simulink model "sim_tanque"  (R2025b)
settings: Solver=VariableStepAuto  StartTime=0.0  StopTime=10.0  RelTol=1e-3
values from neighbouring files (symbols this model uses):
  A = 0.5    [Aula08_lab.m]    (also in Lab10.m; Lab5_6.m; lab3.m; lab4.m)
  g = 9.8    [Aula08_lab.m]    (also in Lab10.m; Lab5_6.m; lab3.m; lab4.m)
  H0 = ((ke*ae0)/(ks*as0*sqrt(2*g)))^2    [Aula08_lab.m]    (also in Lab10.m; Lab5_6.m; lab3.m = H_eq; lab4.m = ((Ke .* ae0) ./ (Ks .* as0 .* sqrt(2*g))).^2)
  Ke = 0.05    [lab3.m]    (also in lab4.m; lab4_bonitinho.m)
  Ks = 0.015    [lab3.m]    (also in lab4.m; lab4_bonitinho.m)
undefined symbols (not defined in the file or in its folder): Ae, As

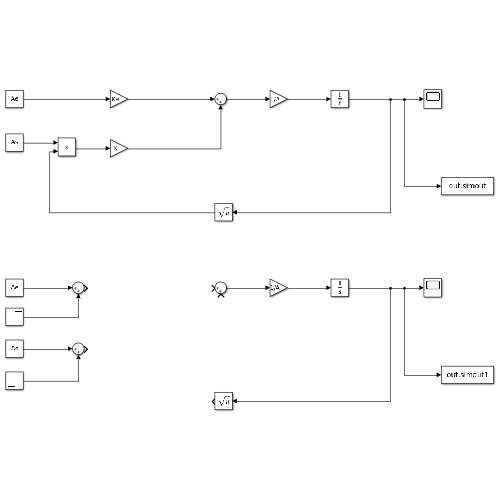
[thumbnail: Simulink's stored preview of the top-level diagram]
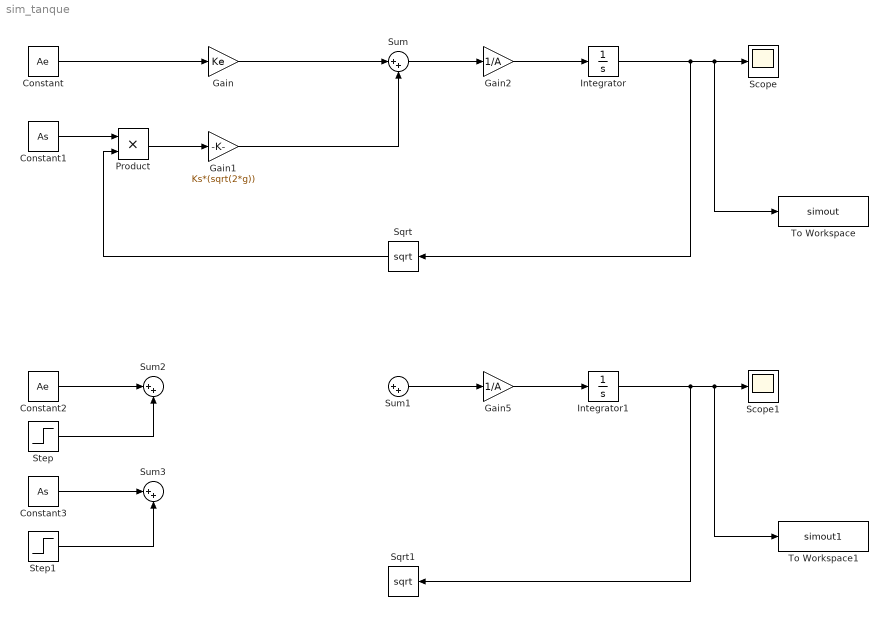
== system sim_tanque ==
  Constant : Constant  Value=Ae
  Constant1 : Constant  Value=As
  Constant2 : Constant  Value=Ae
  Constant3 : Constant  Value=As
  Gain : Gain  Gain=Ke
  Gain1 : Gain  Gain=Ks*(sqrt(2*g))
  Gain2 : Gain  Gain=1/A
  Gain5 : Gain  Gain=1/A
  Integrator : Integrator  InitialCondition=H0
  Integrator1 : Integrator
  Product : Product
  Scope : Scope
  Scope1 : Scope
  Sqrt : Sqrt
  Sqrt1 : Sqrt
  Step : Step  SampleTime=0
  Step1 : Step  SampleTime=0
  Sum{,1..3} (4 alike) : Sum  Inputs=|++
  To Workspace : ToWorkspace  VariableName=simout  SaveFormat=Timeseries  SampleTime=-1
  To Workspace1 : ToWorkspace  VariableName=simout1  SaveFormat=Timeseries  SampleTime=-1
  wires:
  Constant/1 -> Gain/1
  Gain/1 -> Sum/1
  Sum/1 -> Gain2/1
  Gain2/1 -> Integrator/1
  Integrator/1 -> Sqrt/1, To Workspace/1, Scope/1
  Constant1/1 -> Product/1
  Product/1 -> Gain1/1
  Sqrt/1 -> Product/2
  Gain1/1 -> Sum/2
  Gain5/1 -> Integrator1/1
  Sum1/1 -> Gain5/1
  Integrator1/1 -> Sqrt1/1, To Workspace1/1, Scope1/1
  Constant2/1 -> Sum2/1
  Step/1 -> Sum2/2
  Constant3/1 -> Sum3/1
  Step1/1 -> Sum3/2
